simulink model "TP_CFO_Based_PP_pwm_mode"  (R2023b)
settings: Solver=ode4  StartTime=0.0  StopTime=inf  FixedStep=1/500  RelTol=1e-3  EnableMultiTasking=on
values from neighbouring files (symbols this model uses):
  home = [0.45;0;0.49]    [Params.m]
  K1 = [wc1^2,  2*xi1*wc1 - a1_1]    [Params.m]
  K2 = [wc2^2,  2*xi2*wc2 - a1_2]    [Params.m]
  K3 = [wc3^2,  2*xi3*wc3 - a1_3]    [Params.m]
  K4 = [wc4^2,  2*xi4*wc4 - a1_4]    [Params.m]
  pick = [0.66;0;0.3]    [Params.m]
  Place = [-0.425;0.5;0.35]    [Params.m]
undefined symbols (not defined in the file or in its folder): HIL
libraries: quarc_library x6
settings Model: ExtModeTrigDuration=10000  Creator=fvranes  LastModifiedBy=robot
settings SolverCC: AlgebraicLoopSolver=TrustRegion  PositivePriorityOrder=on
settings DataIOCC: ReturnWorkspaceOutputs=off
settings DebuggingCC: UnderspecifiedInitializationDetection=Classic  MergeDetectMultiDrivingBlocksExec=none  UnconnectedInputMsg=warning  UnconnectedOutputMsg=warning  UnconnectedLineMsg=warning
settings ModelReferenceCC: EnableRefExpFcnMdlSchedulingChecks=on  PropagateSignalLabelsOutOfModel=off
settings SFSimCC: CustomCodeUndefinedFunction=UseInterfaceOnly
settings RTWCC: Description=QUARC Win64 Target Using Toolchain  SystemTargetFile=quarc_win64.tlc  Toolchain=QUARC win64 | nmake (64-bit Windows)  BuildConfiguration=Faster Runs
settings STFCustomTargetCC: ConcurrentExecutionCompliant=on  GRTInterface=on  UseToolchainInfoCompliant=on  SystemTargetFile=quarc_win64.tlc
settings GRTTargetCC: ParMdlRefBuildCompliant=off  CompOptLevelCompliant=off  CombineOutputUpdateFcns=off  MatFileLogging=off  CPPClassGenCompliant=off  GRTInterface=on  ExtMode=on  ExtModeMexFile=quarc_comm

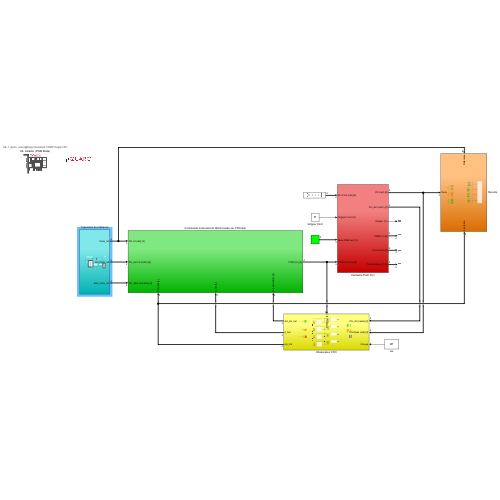
[thumbnail: Simulink's stored preview of the top-level diagram]
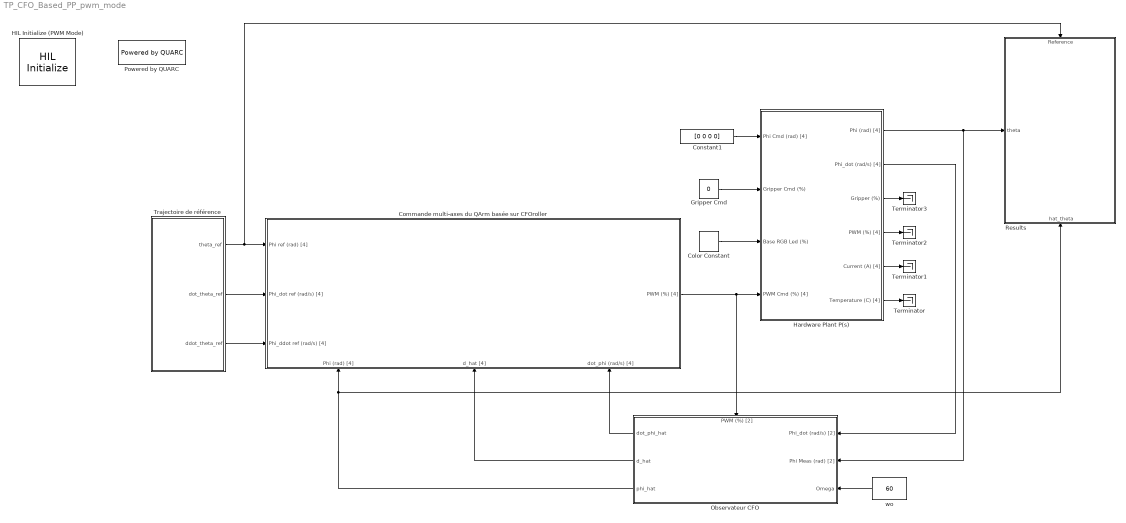
== system TP_CFO_Based_PP_pwm_mode ==
  Color Constant : quarc_library/Sources/Signals/Color Constant  color=[0 1 0]
      settings: SourceProductName=QUARC Targets
  Commande multi-axes du QArm basée sur CFOroller : Subsystem
      settings: PortSchema="{\"entries\":[{\"content\":{\"sides\":[{\"content\":{\"connectorIds\":[\"In1\",\"In2\",\"In3\"]},\"type\":\"ConnectorPlacement.EquallySpacedRectSide\",\"uuid\":\"25f6ea6f-3d46-46f3-9fc0-0185d57d9b43\"},{\"content\":{\"connectorIds\":[\"Out1\"],\"side\":\"RIGHT\"},\"type\":\"ConnectorPlacement.EquallySpacedRectSide\",\"uuid\":\"b6cf073e-ca4c-464e-b4e1-9442ca1008e1\"},{\"content\":{\"side\":\"TOP\"},\"type\":\"ConnectorPlacement.EquallySpacedRectSide\",\"uuid\":\"ffe5b829-7032-4458-83f6-b2e187a076e4\"},{\"content\":{\"connectorIds\":[\"In4\",\"In5\",\"In6\"],\"side\":\"BOTTOM\"},\"type\":\"ConnectorPlacement.EquallySpacedRectSide\",\"uuid\":\"4b5216bb-7b32-4753-9657-18d8be37116d\"}]},\"type\":\"ConnectorPlacement.EquallySpacedConnector\",\"uuid\":\"b7eb2212-47e7-4fcd-9e73-fc098706b9d4\"}],\"packageUris\":[\"http://schema.mathworks.com/mf0/Connector/R2020b\"],\"version\":\"1.0\"}"
  Constant1 : Constant  Value=[0 0 0 0]
  Gripper Cmd : Constant  Value=0
  HIL Initialize (PWM Mode) : quarc_library/Data Acquisition/Generic/Configuration/HIL Initialize  object_name=HIL-1  board_type=qarm_usb  board_number=0@tcpip://localhost:18900?nagle='off'  board_options=j0_mode=1;j1_mode=1;j2_mode=1;j3_mode=1;gripper_mode=0;  exclusive=off  active=on  hardware_clocks=[0]  clock_modes=[]  initial_clock_frequencies=[]  set_clock_params_at_start=off  set_clock_params_at_switch_in=off  set_clock_frequencies_at_start=off  set_clock_frequencies_at_switch_in=off  analog_input_channels=[5:9]  analog_input_configurations=[]  analog_input_maximums=[]  analog_input_minimums=[]  set_analog_input_params_at_start=off  set_analog_input_params_at_switch_in=off  analog_output_channels=[]  analog_output_maximums=inf  analog_output_minimums=-inf  initial_analog_outputs=[0]  final_analog_outputs=[0]  watchdog_analog_outputs=[]  set_analog_output_params_at_start=off  set_analog_output_params_at_switch_in=off  set_analog_outputs_at_start=off  set_analog_outputs_at_switch_in=off  set_analog_outputs_at_terminate=off  set_analog_outputs_at_switch_out=off  set_analog_outputs_on_watchdog=off  digital_input_channels=[]  digital_output_channels=[]  digital_output_configuration=[]  initial_digital_outputs=[0]  final_digital_outputs=[0]  watchdog_digital_outputs=[0]  set_digital_output_params_at_start=off  set_digital_output_params_at_switch_in=off  set_digital_outputs_at_start=off  set_digital_outputs_at_switch_in=off  set_digital_outputs_at_terminate=off  set_digital_outputs_at_switch_out=off  set_digital_outputs_on_watchdog=off  encoder_channels=[]  quadrature=[]  encoder_filter_frequency=[]  initial_encoder_counts=[]  set_encoder_params_at_start=off  set_encoder_params_at_switch_in=off  set_encoder_counts_at_start=off  set_encoder_counts_at_switch_in=off  pwm_channels=[]  pwm_modes=[]  pwm_frequency=[]  pwm_configuration=[]  pwm_alignment=[]  pwm_polarity=[]  pwm_leading_deadband=[]  pwm_trailing_deadband=[]  initial_pwm_outputs=[]  final_pwm_outputs=[]  watchdog_pwm_outputs=[]  set_pwm_params_at_start=off  set_pwm_params_at_switch_in=off  set_pwm_outputs_at_start=off  set_pwm_outputs_at_switch_in=off  set_pwm_outputs_at_terminate=off  set_pwm_outputs_at_switch_out=off  set_pwm_outputs_on_watchdog=off  other_output_channels=[1000:1004 11000:11003 11005:11007]  initial_other_outputs=[zeros(1,9), ones(1,3)]  final_other_outputs=[zeros(1,9), ones(1,3)]  watchdog_other_outputs=zeros(1,12)  set_other_outputs_at_start=off  set_other_outputs_at_switch_in=off  set_other_outputs_at_terminate=on  set_other_outputs_at_switch_out=off  set_other_outputs_on_watchdog=off
  Hardware Plant P(s) : Subsystem
  Observateur CFO : Subsystem
      settings: PortSchema="{\"entries\":[{\"content\":{\"sides\":[{\"content\":{\"connectorIds\":[\"Out1\",\"Out2\",\"Out3\"]},\"type\":\"ConnectorPlacement.EquallySpacedRectSide\",\"uuid\":\"b1ac645d-9d1e-4f6e-bc61-28976872a690\"},{\"content\":{\"connectorIds\":[\"In2\",\"In3\",\"In4\"],\"side\":\"RIGHT\"},\"type\":\"ConnectorPlacement.EquallySpacedRectSide\",\"uuid\":\"7e59dcac-6a8e-4444-81db-3f14db76565a\"},{\"content\":{\"connectorIds\":[\"In1\"],\"side\":\"TOP\"},\"type\":\"ConnectorPlacement.EquallySpacedRectSide\",\"uuid\":\"ce092a22-ec44-4e1c-8718-a0a100faa11b\"}]},\"type\":\"ConnectorPlacement.EquallySpacedConnector\",\"uuid\":\"dc8234ad-9229-4c64-a6ff-80b8db3f41cc\"}],\"packageUris\":[\"http://schema.mathworks.com/mf0/Connector/R2020b\"],\"version\":\"1.0\"}"
  Powered by QUARC : quarc_library/Logos/Powered by QUARC
  Results : Subsystem
      settings: PortSchema="{\"entries\":[{\"content\":{\"sides\":[{\"content\":{\"connectorIds\":[\"In1\"]},\"type\":\"ConnectorPlacement.EquallySpacedRectSide\",\"uuid\":\"fa6fdd80-9ba7-487b-8585-3ea4afe8c15a\"},{\"content\":{\"side\":\"RIGHT\"},\"type\":\"ConnectorPlacement.EquallySpacedRectSide\",\"uuid\":\"3312bcac-8289-413d-bf87-6a8d7db3217e\"},{\"content\":{\"connectorIds\":[\"In2\"],\"side\":\"TOP\"},\"type\":\"ConnectorPlacement.EquallySpacedRectSide\",\"uuid\":\"0731ee27-fa4b-422b-b333-a0e403238348\"},{\"content\":{\"connectorIds\":[\"In3\"],\"side\":\"BOTTOM\"},\"type\":\"ConnectorPlacement.EquallySpacedRectSide\",\"uuid\":\"d410c791-6845-40d9-b869-911e609371ee\"}]},\"type\":\"ConnectorPlacement.EquallySpacedConnector\",\"uuid\":\"747f7da3-1a68-4a17-a06e-f94e78aaaccb\"}],\"packageUris\":[\"http://schema.mathworks.com/mf0/Connector/R2020b\"],\"version\":\"1.0\"}"
  Terminator{,1..3} (4 alike) : Terminator
  Trajectoire de référence : Subsystem
  wo : Constant  Value=60
  wires:
  Color Constant/1 -> Hardware Plant P(s)/3(Base RGB Led (%))
  Hardware Plant P(s)/1(Phi (rad) [4]) -> Observateur CFO/3(Phi Meas (rad) [2]), Results/1(theta)
  Commande multi-axes du QArm basée sur CFOroller/1(PWM (%) [4]) -> Observateur CFO/1(PWM (%) [2]), Hardware Plant P(s)/4(PWM Cmd (%) [4])
  Constant1/1 -> Hardware Plant P(s)/1(Phi Cmd (rad) [4])
  wo/1 -> Observateur CFO/4(Omega)
  Trajectoire de référence/1(theta_ref) -> Commande multi-axes du QArm basée sur CFOroller/1(Phi ref (rad) [4]), Results/2(Reference)
  Trajectoire de référence/3(ddot_theta_ref) -> Commande multi-axes du QArm basée sur CFOroller/3(Phi_ddot ref (rad/s) [4])
  Trajectoire de référence/2(dot_theta_ref) -> Commande multi-axes du QArm basée sur CFOroller/2(Phi_dot ref (rad/s) [4])
  Hardware Plant P(s)/6(Temperature (C) [4]) -> Terminator/1
  Hardware Plant P(s)/5(Current (A) [4]) -> Terminator1/1
  Hardware Plant P(s)/4(PWM (%) [4]) -> Terminator2/1
  Hardware Plant P(s)/3(Gripper (%)) -> Terminator3/1
  Hardware Plant P(s)/2(Phi_dot (rad/s) [4]) -> Observateur CFO/2(Phi_dot (rad/s) [2])
  Gripper Cmd/1 -> Hardware Plant P(s)/2(Gripper Cmd (%))
  Observateur CFO/1(dot_phi_hat) -> Commande multi-axes du QArm basée sur CFOroller/6(dot_phi (rad/s) [4])
  Observateur CFO/2("d_hat ") -> Commande multi-axes du QArm basée sur CFOroller/5(d_hat [4])
  Observateur CFO/3(phi_hat) -> Commande multi-axes du QArm basée sur CFOroller/4(Phi (rad) [4]), Results/3(hat_theta)

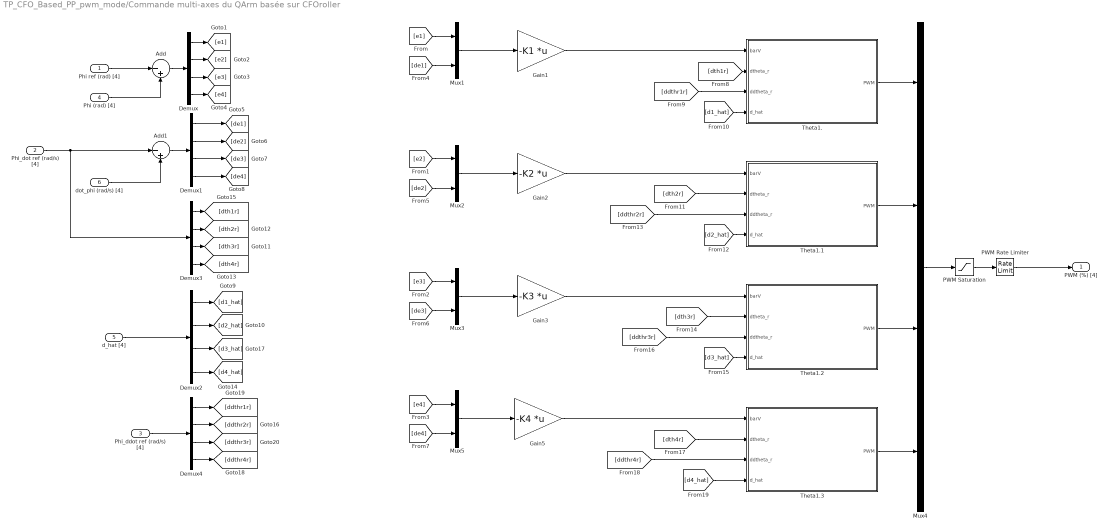
== system TP_CFO_Based_PP_pwm_mode/Commande multi-axes du QArm basée sur CFOroller ==
  Phi ref (rad) [4] : Inport
  Phi_dot ref (rad/s) [4] : Inport  Port=2
  Phi_ddot ref (rad/s) [4] : Inport  Port=3
  Phi (rad) [4] : Inport  Port=4
  d_hat [4] : Inport  Port=5
  dot_phi (rad/s) [4] : Inport  Port=6
  Add : Sum  Inputs=|-+
  Add1 : Sum  Inputs=|-+
  Demux{,1..4} (5 alike) : Demux
  Gain1 : Gain  Gain=-K1  Multiplication=Matrix(K*u)
  Gain2 : Gain  Gain=-K2  Multiplication=Matrix(K*u)
  Gain3 : Gain  Gain=-K3  Multiplication=Matrix(K*u)
  Gain5 : Gain  Gain=-K4  Multiplication=Matrix(K*u)
  Mux{1..3,5} (4 alike) : Mux  Inputs=2
  Mux4 : Mux
  PWM Rate Limiter : RateLimiter  RisingSlewLimit=0.5*[2 2 2 2]  FallingSlewLimit=0.5*[-2 -2 -2 -2]  SampleTimeMode=inherited
  PWM Saturation : Saturate  UpperLimit=[1 1 1 1]  LowerLimit=[-1 -1 -1 -1]
  Theta1. : MATLAB Function  TreatAsAtomicUnit=on
  Theta1.1 : MATLAB Function  TreatAsAtomicUnit=on
  Theta1.2 : MATLAB Function  TreatAsAtomicUnit=on
  Theta1.3 : MATLAB Function  TreatAsAtomicUnit=on
  PWM (%) [4] : Outport  VectorParamsAs1DForOutWhenUnconnected=off
  wires:
  PWM Saturation/1 -> PWM Rate Limiter/1
  PWM Rate Limiter/1 -> PWM (%) [4]/1
  [e1] -> Mux1/1
  Add1/1 -> Demux1/1
  Phi (rad) [4]/1 -> Add/2
  Phi_ddot ref (rad/s) [4]/1 -> Demux4/1
  [e2] -> Mux2/1
  [de2] -> Mux2/2
  Phi_dot ref (rad/s) [4]/1 -> Demux3/1, Add1/1
  [d2_hat] -> Theta1.1/4(d_hat)
  dot_phi (rad/s) [4]/1 -> Add1/2
  [de1] -> Mux1/2
  Add/1 -> Demux/1
  Phi ref (rad) [4]/1 -> Add/1
  Mux4/1 -> PWM Saturation/1
  d_hat [4]/1 -> Demux2/1
  [d1_hat] -> Theta1./4(d_hat)
  Theta1./1(PWM) -> Mux4/1
  Theta1.1/1(PWM) -> Mux4/2
  Demux/1 -> [e1]
  Demux/2 -> [e2]
  Demux3/1 -> [dth1r]
  Demux3/2 -> [dth2r]
  Demux2/1 -> [d1_hat]
  Demux2/2 -> [d2_hat]
  Demux4/1 -> [ddthr1r]
  Demux4/2 -> [ddthr2r]
  Demux/3 -> [e3]
  Demux/4 -> [e4]
  Demux1/1 -> [de1]
  Demux1/2 -> [de2]
  Demux1/3 -> [de3]
  Demux1/4 -> [de4]
  Demux3/3 -> [dth3r]
  Demux3/4 -> [dth4r]
  Demux2/3 -> [d3_hat]
  Demux2/4 -> [d4_hat]
  Demux4/3 -> [ddthr3r]
  Demux4/4 -> [ddthr4r]
  Theta1.3/1(PWM) -> Mux4/4
  Theta1.2/1(PWM) -> Mux4/3
  [d3_hat] -> Theta1.2/4(d_hat)
  [de3] -> Mux3/2
  [de4] -> Mux5/2
  [e4] -> Mux5/1
  [e3] -> Mux3/1
  [dth1r] -> Theta1./2(dtheta_r)
  [ddthr1r] -> Theta1./3(ddtheta_r)
  [dth2r] -> Theta1.1/2(dtheta_r)
  [ddthr2r] -> Theta1.1/3(ddtheta_r)
  [dth3r] -> Theta1.2/2(dtheta_r)
  [ddthr3r] -> Theta1.2/3(ddtheta_r)
  [dth4r] -> Theta1.3/2(dtheta_r)
  [ddthr4r] -> Theta1.3/3(ddtheta_r)
  [d4_hat] -> Theta1.3/4(d_hat)
  Gain1/1 -> Theta1./1(barV)
  Gain2/1 -> Theta1.1/1(barV)
  Gain3/1 -> Theta1.2/1(barV)
  Gain5/1 -> Theta1.3/1(barV)
  Mux5/1 -> Gain5/1
  Mux3/1 -> Gain3/1
  Mux2/1 -> Gain2/1
  Mux1/1 -> Gain1/1

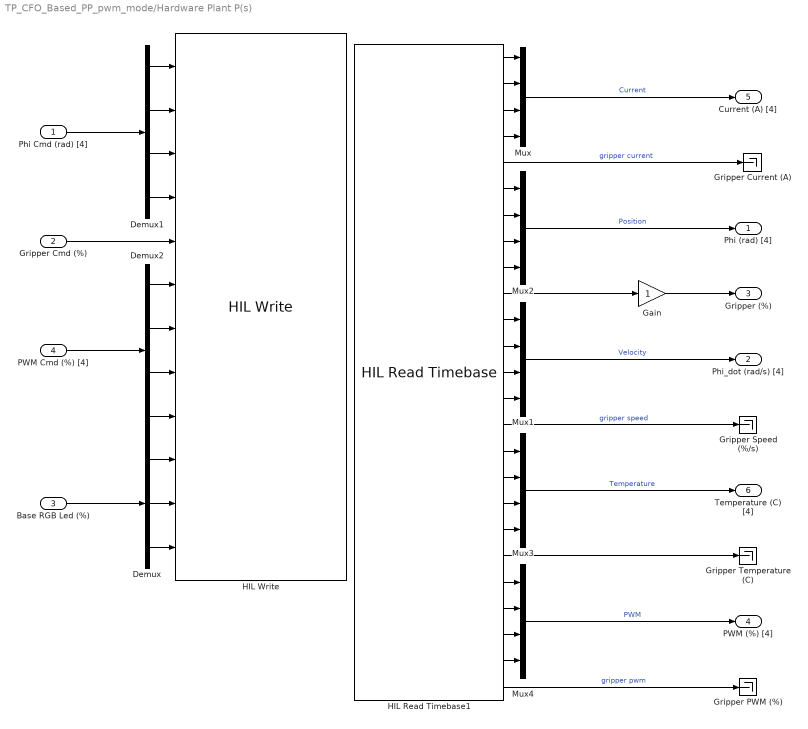
== system TP_CFO_Based_PP_pwm_mode/Hardware Plant P(s) ==
  Phi Cmd (rad) [4] : Inport
  Gripper Cmd (%) : Inport  Port=2
  Base RGB Led (%) : Inport  Port=3
  PWM Cmd (%) [4] : Inport  Port=4
  Demux : Demux  Outputs=3
  Demux1 : Demux
  Demux2 : Demux
  Gain : Gain
  Gripper Current (A) : Terminator
  Gripper PWM (%) : Terminator
  Gripper Speed (%/s) : Terminator
  Gripper Temperature (C) : Terminator
  HIL Read Timebase1 : quarc_library/Data Acquisition/Generic/Timebases/HIL Read Timebase  object_name=HIL-1  clock=0  analog_channels=[5:9]  encoder_channels=[]  digital_channels=[]  other_channels=[1000:1004 3000:3004 10000:10004 11000:11004]  active=on  vector_output=off  data_type_mode=Inherit via back propagation  encoder_data_type=double  digital_data_type=boolean  overflow_mode=Synchronize (for simulated cards only)  samples_in_buffer=1
  HIL Write : quarc_library/Data Acquisition/Generic/Immediate I//O/HIL Write  object_name=HIL-1  analog_channels=[]  pwm_channels=[]  digital_channels=[]  other_channels=[1000:1004 11000:11003 11005:11007]  sample_time=-1  active=on  vector_input=off
  Mux{,1..4} (5 alike) : Mux
  Phi (rad) [4] : Outport  VectorParamsAs1DForOutWhenUnconnected=off
  Phi_dot (rad/s) [4] : Outport  Port=2  VectorParamsAs1DForOutWhenUnconnected=off
  Gripper (%) : Outport  Port=3  VectorParamsAs1DForOutWhenUnconnected=off
  PWM (%) [4] : Outport  Port=4  VectorParamsAs1DForOutWhenUnconnected=off
  Current (A) [4] : Outport  Port=5  VectorParamsAs1DForOutWhenUnconnected=off
  Temperature (C) [4] : Outport  Port=6  VectorParamsAs1DForOutWhenUnconnected=off
  wires:
  HIL Read Timebase1/14 -> Mux1/4
  HIL Read Timebase1/9 -> Mux2/4
  HIL Read Timebase1/6 -> Mux2/1
  HIL Read Timebase1/18 -> Mux3/3
  HIL Read Timebase1/8 -> Mux2/3
  HIL Read Timebase1/12 -> Mux1/2
  HIL Read Timebase1/4 -> Mux/4
  HIL Read Timebase1/7 -> Mux2/2
  HIL Read Timebase1/5 -> Gripper Current (A)/1  "gripper current"
  HIL Read Timebase1/15 -> Gripper Speed (%/s)/1  "gripper speed"
  Demux/3 -> HIL Write/12
  HIL Read Timebase1/3 -> Mux/3
  HIL Read Timebase1/17 -> Mux3/2
  HIL Read Timebase1/16 -> Mux3/1
  HIL Read Timebase1/11 -> Mux1/1
  Demux/1 -> HIL Write/10
  HIL Read Timebase1/19 -> Mux3/4
  Demux/2 -> HIL Write/11
  HIL Read Timebase1/13 -> Mux1/3
  HIL Read Timebase1/2 -> Mux/2
  HIL Read Timebase1/1 -> Mux/1
  HIL Read Timebase1/20 -> Gripper Temperature (C)/1
  Mux/1 -> Current (A) [4]/1  "Current"
  Mux1/1 -> Phi_dot (rad/s) [4]/1  "Velocity"
  Mux3/1 -> Temperature (C) [4]/1  "Temperature"
  Base RGB Led (%)/1 -> Demux/1
  Demux1/1 -> HIL Write/1
  Demux1/2 -> HIL Write/2
  Demux1/3 -> HIL Write/3
  Demux1/4 -> HIL Write/4
  Phi Cmd (rad) [4]/1 -> Demux1/1
  PWM Cmd (%) [4]/1 -> Demux2/1
  Demux2/1 -> HIL Write/6
  Demux2/2 -> HIL Write/7
  Demux2/3 -> HIL Write/8
  Demux2/4 -> HIL Write/9
  Mux2/1 -> Phi (rad) [4]/1  "Position"
  HIL Read Timebase1/21 -> Mux4/1
  HIL Read Timebase1/22 -> Mux4/2
  HIL Read Timebase1/23 -> Mux4/3
  HIL Read Timebase1/24 -> Mux4/4
  HIL Read Timebase1/25 -> Gripper PWM (%)/1  "gripper pwm"
  Mux4/1 -> PWM (%) [4]/1  "PWM"
  HIL Read Timebase1/10 -> Gain/1
  Gain/1 -> Gripper (%)/1
  Gripper Cmd (%)/1 -> HIL Write/5

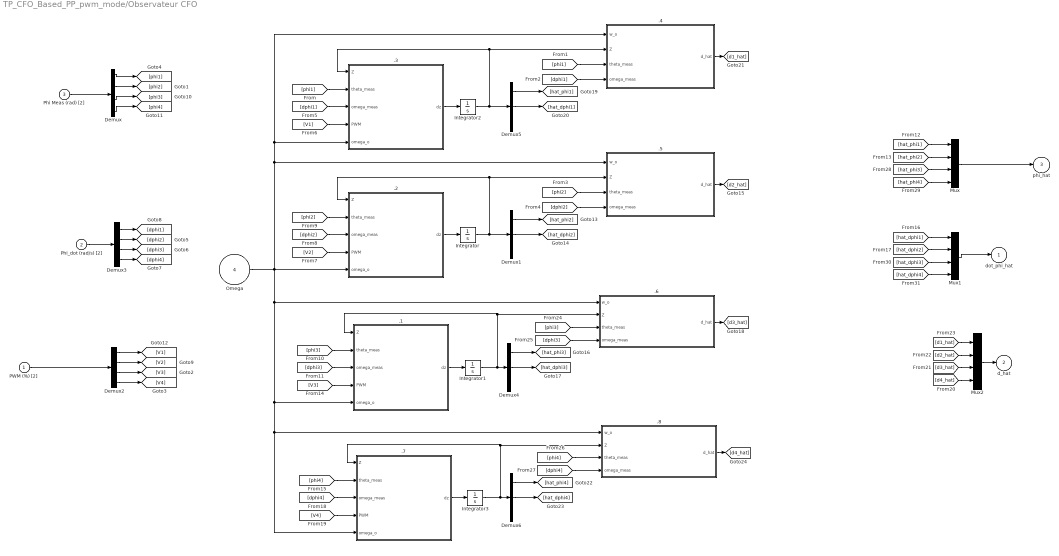
== system TP_CFO_Based_PP_pwm_mode/Observateur CFO ==
  PWM (%) [2] : Inport
  Phi_dot (rad/s) [2] : Inport  Port=2
  Phi Meas (rad) [2] : Inport  Port=3
  Omega : Inport  Port=4
  .1 : MATLAB Function  TreatAsAtomicUnit=on
  .2 : MATLAB Function  TreatAsAtomicUnit=on
  .3 : MATLAB Function  TreatAsAtomicUnit=on
  .4 : MATLAB Function  TreatAsAtomicUnit=on
  .5 : MATLAB Function  TreatAsAtomicUnit=on
  .6 : MATLAB Function  TreatAsAtomicUnit=on
  .7 : MATLAB Function  TreatAsAtomicUnit=on
  .8 : MATLAB Function  TreatAsAtomicUnit=on
  Demux : Demux
  Demux{1,4..6} (4 alike) : Demux  Outputs=3
  Demux2 : Demux
  Demux3 : Demux
  Integrator : Integrator  InitialCondition=[3.5*10^-3 0 0]
  Integrator1 : Integrator  InitialCondition=[5*10^-3 0 0]
  Integrator2 : Integrator  InitialCondition=[0 0 0]
  Integrator3 : Integrator  InitialCondition=[0 0 0]
  Mux : Mux
  Mux1 : Mux
  Mux2 : Mux
  dot_phi_hat : Outport
  "d_hat " : Outport  Port=2
  phi_hat : Outport  Port=3
  wires:
  .2/1(dz) -> Integrator/1
  Integrator/1 -> .5/2(Z), .2/1(Z), Demux1/1
  [V2] -> .2/4(PWM)
  Phi Meas (rad) [2]/1 -> Demux/1
  Phi_dot (rad/s) [2]/1 -> Demux3/1
  Demux/1 -> [phi1]
  Demux/2 -> [phi2]
  Demux3/1 -> [dphi1]
  Demux3/2 -> [dphi2]
  Demux2/1 -> [V1]
  Demux2/2 -> [V2]
  [phi2] -> .2/2(theta_meas)
  [dphi2] -> .2/3(omega_meas)
  Demux1/1 -> [hat_phi2]
  Demux1/2 -> [hat_dphi2]
  [dphi3] -> .1/3(omega_meas)
  [phi3] -> .1/2(theta_meas)
  [V3] -> .1/4(PWM)
  Integrator1/1 -> .1/1(Z), .6/2(Z), Demux4/1
  .1/1(dz) -> Integrator1/1
  Mux/1 -> phi_hat/1
  Mux1/1 -> dot_phi_hat/1
  Mux2/1 -> "d_hat "/1
  [hat_phi1] -> Mux/1
  [hat_phi2] -> Mux/2
  [hat_dphi1] -> Mux1/1
  [hat_dphi2] -> Mux1/2
  [d1_hat] -> Mux2/1
  [d2_hat] -> Mux2/2
  Demux4/1 -> [hat_phi3]
  Demux4/2 -> [hat_dphi3]
  [phi2] -> .5/3(theta_meas)
  [dphi2] -> .5/4(omega_meas)
  .5/1(d_hat) -> [d2_hat]
  [phi3] -> .6/3(theta_meas)
  [dphi3] -> .6/4(omega_meas)
  .6/1(d_hat) -> [d3_hat]
  Demux2/4 -> [V4]
  Demux2/3 -> [V3]
  Demux3/3 -> [dphi3]
  Demux3/4 -> [dphi4]
  Demux/3 -> [phi3]
  Demux/4 -> [phi4]
  .4/1(d_hat) -> [d1_hat]
  Omega/1 -> .4/1(w_o), .3/5(omega_o), .5/1(w_o), .2/5(omega_o), .6/1(w_o), .7/5(omega_o), .8/1(w_o), .1/5(omega_o)
  Demux5/2 -> [hat_dphi1]
  Demux5/1 -> [hat_phi1]
  [dphi1] -> .3/3(omega_meas)
  [phi1] -> .3/2(theta_meas)
  [V1] -> .3/4(PWM)
  Integrator2/1 -> Demux5/1, .3/1(Z), .4/2(Z)
  .3/1(dz) -> Integrator2/1
  .8/1(d_hat) -> [d4_hat]
  [dphi4] -> .8/4(omega_meas)
  [phi4] -> .8/3(theta_meas)
  Demux6/2 -> [hat_dphi4]
  Demux6/1 -> [hat_phi4]
  .7/1(dz) -> Integrator3/1
  Integrator3/1 -> Demux6/1, .8/2(Z), .7/1(Z)
  [V4] -> .7/4(PWM)
  [phi4] -> .7/2(theta_meas)
  [dphi4] -> .7/3(omega_meas)
  [d3_hat] -> Mux2/3
  [d4_hat] -> Mux2/4
  [hat_phi3] -> Mux/3
  [hat_phi4] -> Mux/4
  [hat_dphi3] -> Mux1/3
  [hat_dphi4] -> Mux1/4
  PWM (%) [2]/1 -> Demux2/1
  [phi1] -> .4/3(theta_meas)
  [dphi1] -> .4/4(omega_meas)

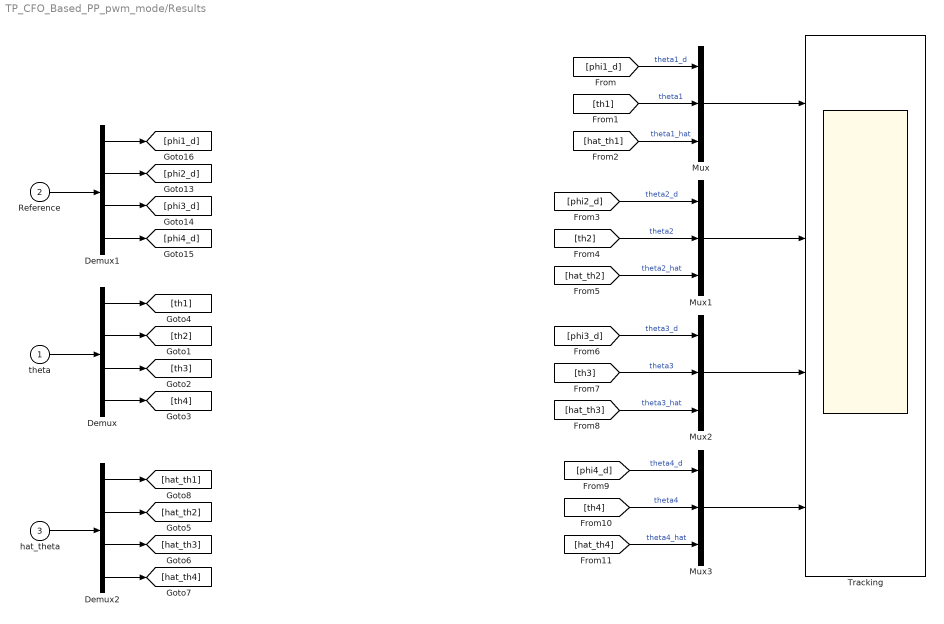
== system TP_CFO_Based_PP_pwm_mode/Results ==
  theta : Inport
  Reference : Inport  Port=2
  hat_theta : Inport  Port=3
  Demux : Demux
  Demux1 : Demux
  Demux2 : Demux
  Mux{,1..3} (4 alike) : Mux  Inputs=3
  Tracking : Scope  NumInputPorts=4
  wires:
  Mux/1 -> Tracking/1
  Demux/3 -> [th3]
  theta/1 -> Demux/1
  Demux/4 -> [th4]
  Demux/2 -> [th2]
  Demux/1 -> [th1]
  Demux1/1 -> [phi1_d]
  Demux1/2 -> [phi2_d]
  Demux1/4 -> [phi4_d]
  Reference/1 -> Demux1/1
  Demux1/3 -> [phi3_d]
  Demux2/1 -> [hat_th1]
  Demux2/2 -> [hat_th2]
  Demux2/4 -> [hat_th4]
  hat_theta/1 -> Demux2/1
  Demux2/3 -> [hat_th3]
  [phi1_d] -> Mux/1  "theta1_d"
  [th1] -> Mux/2  "theta1"
  [hat_th1] -> Mux/3  "theta1_hat"
  Mux1/1 -> Tracking/2
  Mux2/1 -> Tracking/3
  Mux3/1 -> Tracking/4
  [phi2_d] -> Mux1/1  "theta2_d"
  [th2] -> Mux1/2  "theta2"
  [hat_th2] -> Mux1/3  "theta2_hat"
  [phi3_d] -> Mux2/1  "theta3_d"
  [th3] -> Mux2/2  "theta3"
  [hat_th3] -> Mux2/3  "theta3_hat"
  [phi4_d] -> Mux3/1  "theta4_d"
  [th4] -> Mux3/2  "theta4"
  [hat_th4] -> Mux3/3  "theta4_hat"

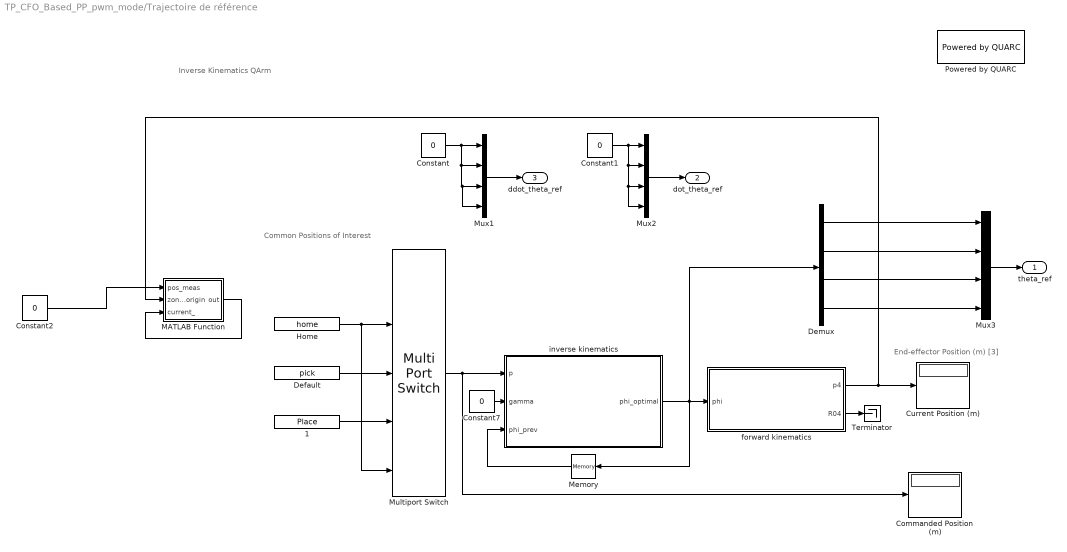
== system TP_CFO_Based_PP_pwm_mode/Trajectoire de référence ==
  note: Inverse Kinematics
      | QArm
  note: End-effector
      | Position (m) [3]
  note: Common Positions of Interest
  1 : Constant  Value=Place
  Commanded Position (m) : Display
  Constant{,1..2,7} (4 alike) : Constant  Value=0
  Current Position (m) : Display
  Default : Constant  Value=pick
  Demux : Demux
  Home : Constant  Value=home
  MATLAB Function : MATLAB Function  TreatAsAtomicUnit=on
  Memory : Memory  InitialCondition=[0 0 0 0]
  Multiport Switch : MultiPortSwitch  DataPortForDefault=Additional data port  SaturateOnIntegerOverflow=off  InputSameDT=off
  Mux1 : Mux
  Mux2 : Mux
  Mux3 : Mux
  Powered by QUARC : quarc_library/Logos/Powered by QUARC
  Terminator : Terminator
  forward kinematics : MATLAB Function  TreatAsAtomicUnit=on
  inverse kinematics : MATLAB Function  TreatAsAtomicUnit=on
  theta_ref : Outport
  dot_theta_ref : Outport  Port=2
  ddot_theta_ref : Outport  Port=3
  wires:
  Constant/1 -> Mux1/4, Mux1/3, Mux1/2, Mux1/1
  Constant1/1 -> Mux2/4, Mux2/3, Mux2/2, Mux2/1
  Mux2/1 -> dot_theta_ref/1
  Mux1/1 -> ddot_theta_ref/1
  Constant7/1 -> inverse kinematics/2(gamma)
  inverse kinematics/1(phi_optimal) -> Demux/1, Memory/1, forward kinematics/1(phi)
  1/1 -> Multiport Switch/4
  Multiport Switch/1 -> Commanded Position (m)/1, inverse kinematics/1(p)
  forward kinematics/1(p4) -> MATLAB Function/2(zone_origin), Current Position (m)/1
  Home/1 -> Multiport Switch/5, Multiport Switch/2
  Default/1 -> Multiport Switch/3
  forward kinematics/2(R04) -> Terminator/1
  Memory/1 -> inverse kinematics/3(phi_prev)
  Demux/1 -> Mux3/1
  Demux/4 -> Mux3/4
  Demux/3 -> Mux3/3
  Demux/2 -> Mux3/2
  Mux3/1 -> theta_ref/1
  Constant2/1 -> MATLAB Function/1(pos_meas)
  MATLAB Function/1(out) -> MATLAB Function/3(current_)

== matlab function TP_CFO_Based_PP_pwm_mode/Observateur CFO/.5 ==
  data: w_o input; Z input; theta_meas input; omega_meas input; d_hat output
function d_hat  = tau_tot_hat_joint1(w_o,Z, theta_meas, omega_meas)


z1 = Z(1); z2 = Z(2); z3 = Z(3);


%% Erreurs d'observation
e_theta = theta_meas - z1;
e_omega = omega_meas - z2;

%% Gains CFO
l1 = 9*w_o;
l2 = 12*w_o*w_o;

%% Terme de correction
Le = l2*e_theta + l1*e_omega;

d_hat = Le + z3;
end

== matlab function TP_CFO_Based_PP_pwm_mode/Observateur CFO/.6 ==
  data: w_o input; Z input; theta_meas input; omega_meas input; d_hat output
function d_hat = d_hat_joint3(w_o, Z, theta_meas, omega_meas)

z1 = Z(1);
z2 = Z(2);
z3 = Z(3);



%% Erreurs d'observation
e_theta = theta_meas - z1;
e_omega = omega_meas - z2;

%% Gains CFO
l1 = 9*w_o;
l2 = 12*w_o*w_o;

%% Terme de correction
Le = l2*e_theta + l1*e_omega;

d_hat = Le + z3;
end

== matlab function TP_CFO_Based_PP_pwm_mode/Observateur CFO/.3 ==
  data: Z input; theta_meas input; omega_meas input; PWM input; dz output; omega_o input
function dz = cfo_obs_joint1(Z, theta_meas, omega_meas, PWM, omega_o)

% CFO - Joint 1
V = 12*PWM;
%% Etats observateur
z1 = Z(1);      % theta_hat
z2 = Z(2);      % omega_hat
z3 = Z(3);      % etat interne CFO

%% Parametres Joint 1
a0 = 23.4652;
a1 = 91.4161;

%% Erreurs d'observation
e_theta = theta_meas - z1;
e_omega = omega_meas - z2;

%% Gains CFO
l1 = 9*omega_o;
l2 = 12*omega_o*omega_o;
lambda = (4/3)*omega_o;

%% Terme de correction
Le = l2*e_theta + l1*e_omega;

%% Dynamique CFO
theta_point_hat = z2;
omega_point_hat = -a1*z2+a0*V+Le+z3;
z3_point = lambda * Le;

%% Sortie
dz = [theta_point_hat omega_point_hat z3_point];


end

== matlab function TP_CFO_Based_PP_pwm_mode/Observateur CFO/.4 ==
  data: w_o input; Z input; theta_meas input; omega_meas input; d_hat output
function d_hat = d_hat_joint2(w_o, Z, theta_meas, omega_meas)

z1 = Z(1);
z2 = Z(2);
z3 = Z(3);

%% Erreurs d'observation
e_theta = theta_meas - z1;
e_omega = omega_meas - z2;

%% Gains CFO
l1 = 9*w_o;
l2 = 12*w_o*w_o;

%% Terme de correction
Le = l2*e_theta + l1*e_omega;

d_hat = Le + z3;
end

== matlab function TP_CFO_Based_PP_pwm_mode/Observateur CFO/.7 ==
  data: Z input; theta_meas input; omega_meas input; PWM input; dz output; omega_o input
function dz = cfo_obs_joint4(Z, theta_meas, omega_meas, PWM, omega_o)

z1 = Z(1);
z2 = Z(2);
z3 = Z(3);

% Parametres locaux Joint 4
a0 = 271.48313954;
a1 = 671.78502879;

% PWM -> tension
V = 12*PWM;

%% Erreurs d'observation
e_theta = theta_meas - z1;
e_omega = omega_meas - z2;

%% Gains CFO
l1 = 9*omega_o;
l2 = 12*omega_o*omega_o;
lambda = (4/3)*omega_o;

%% Terme de correction
Le = l2*e_theta + l1*e_omega;

%% Dynamique CFO
theta_point_hat = z2;
omega_point_hat = -a1*z2+a0*V+Le+z3;
z3_point = lambda * Le;

%% Sortie
dz = [theta_point_hat omega_point_hat z3_point];


end

== matlab function TP_CFO_Based_PP_pwm_mode/Observateur CFO/.2 ==
  data: Z input; theta_meas input; omega_meas input; PWM input; dz output; omega_o input
function dz = cfo_obs_joint2(Z, theta_meas, omega_meas, PWM, omega_o)

z1 = Z(1);
z2 = Z(2);
z3 = Z(3);

% Parametres locaux Joint 2
a0 = 17.59887839;
a1 = 68.11562089;

% PWM -> tension
V = 12*PWM;

%% Erreurs d'observation
e_theta = theta_meas - z1;
e_omega = omega_meas - z2;

%% Gains CFO
l1 = 9*omega_o;
l2 = 12*omega_o*omega_o;
lambda = (4/3)*omega_o;

%% Terme de correction
Le = l2*e_theta + l1*e_omega;

%% Dynamique CFO
theta_point_hat = z2;
omega_point_hat = -a1*z2+a0*V+Le+z3;
z3_point = lambda * Le;

%% Sortie
dz = [theta_point_hat omega_point_hat z3_point];


end

== matlab function TP_CFO_Based_PP_pwm_mode/Observateur CFO/.8 ==
  data: w_o input; Z input; theta_meas input; omega_meas input; d_hat output
function d_hat = d_hat_joint4(w_o, Z, theta_meas, omega_meas)

z1 = Z(1);
z2 = Z(2);
z3 = Z(3);

%% Erreurs d'observation
e_theta = theta_meas - z1;
e_omega = omega_meas - z2;

%% Gains CFO
l1 = 9*w_o;
l2 = 12*w_o*w_o;

%% Terme de correction
Le = l2*e_theta + l1*e_omega;

d_hat = Le + z3;
end

== matlab function TP_CFO_Based_PP_pwm_mode/Commande multi-axes du QArm basée sur CFOroller/Theta1.1 ==
  data: barV input; dtheta_r input; ddtheta_r input; PWM output; d_hat input
function PWM = joint2_control(barV, dtheta_r, ddtheta_r, d_hat)

a0 = 17.59887839;
a1 = 68.11562089;

V = (barV-d_hat+a1*dtheta_r+ddtheta_r)/(a0);

% Saturation 
if V > 12
    V = 12;
elseif V < -12
    V = -12;
end

% Tension -> PWM
PWM = V/12;

end

== matlab function TP_CFO_Based_PP_pwm_mode/Commande multi-axes du QArm basée sur CFOroller/Theta1.2 ==
  data: barV input; dtheta_r input; ddtheta_r input; PWM output; d_hat input
function PWM = joint3_control(barV, dtheta_r, ddtheta_r, d_hat)

a0 = 23.46517119;
a1 = 93.20178023;

V = (barV-d_hat+a1*dtheta_r+ddtheta_r)/(a0);

if V > 12
    V = 12;
elseif V < -12
    V = -12;
end

PWM = V/12;

end

== matlab function TP_CFO_Based_PP_pwm_mode/Commande multi-axes du QArm basée sur CFOroller/Theta1. ==
  data: barV input; dtheta_r input; ddtheta_r input; PWM output; d_hat input
function PWM = joint1_control(barV, dtheta_r, ddtheta_r, d_hat)

%% Parametres Joint 1
a0 = 23.46517119;
a1 = 91.41606594;

%% Tension moteur
V = (barV-d_hat+a1*dtheta_r+ddtheta_r)/(a0);

%% Saturation 
if V > 12
    V = 12;
elseif V < -12
    V = -12;
end

%% Conversion tension -> PWM normalise
PWM = V/12;

end

== matlab function TP_CFO_Based_PP_pwm_mode/Commande multi-axes du QArm basée sur CFOroller/Theta1.3 ==
  data: barV input; dtheta_r input; ddtheta_r input; PWM output; d_hat input
function PWM = joint4_control(barV, dtheta_r, ddtheta_r, d_hat)

a0 = 271.48313954;
a1 = 671.78502879;

V = (barV-d_hat+a1*dtheta_r+ddtheta_r)/(a0);

if V > 12
    V = 12;
elseif V < -12
    V = -12;
end

PWM = V/12;

end

== matlab function TP_CFO_Based_PP_pwm_mode/Observateur CFO/.1 ==
  data: Z input; theta_meas input; omega_meas input; PWM input; dz output; omega_o input
function dz = cfo_obs_joint3(Z, theta_meas, omega_meas, PWM, omega_o)

z1 = Z(1);
z2 = Z(2);
z3 = Z(3);

% Parametres Joint 3
a0 = 23.46517119;
a1 = 93.20178023;

% PWM -> tension
V = 12*PWM;

%% Erreurs d'observation
e_theta = theta_meas - z1;
e_omega = omega_meas - z2;

%% Gains CFO
l1 = 9*omega_o;
l2 = 12*omega_o*omega_o;
lambda = (4/3)*omega_o;

%% Terme de correction
Le = l2*e_theta + l1*e_omega;

%% Dynamique CFO
theta_point_hat = z2;
omega_point_hat = -a1*z2+a0*V+Le+z3;
z3_point = lambda * Le;

%% Sortie
dz = [theta_point_hat omega_point_hat z3_point];
end

== matlab function TP_CFO_Based_PP_pwm_mode/Trajectoire de référence/forward kinematics ==
  data: phi input; p4 output; R04 output
function [p4, R04] = qarmForwardKinematics(phi)

%% QUANSER_ARM_FPK
% v 4.0 - 4th June 2020

% REFERENCE: 
% Chapter 3. Forward Kinematics
% Robot Dynamics and Control 
% Spong, Vidyasagar
% 1989

% INPUTS:
% phi     : Alternate joint angles vector 4 x 1

% OUTPUTS:
% p4      : End-effector frame {4} position vector expressed in base frame {0}
% R04     : rotation matrix from end-effector frame {4} to base frame {0}

%% Manipulator parameters:
L1 = 0.1400;
L2 = 0.3500;
L3 = 0.0500;
L4 = 0.2500;
L5 = 0.1500;

%% Alternate parameters
l1 = L1;
l2 = sqrt(L2^2 + L3^2);
l3 = L4 + L5;
beta = atan(L3/L2);

%% From phi space to theta space 
theta = phi;
theta(1) = phi(1);
theta(2) = phi(2) + beta - pi/2;
theta(3) = phi(3) - beta;
theta(4) = phi(4);

%% Transformation matrices for all frames:

% T{i-1}{i} = quanser_arm_DH(  a, alpha,  d,     theta );
        T01 = quanser_arm_DH(  0, -pi/2, l1,  theta(1) );
        T12 = quanser_arm_DH( l2,     0,  0,  theta(2) );
        T23 = quanser_arm_DH(  0, -pi/2,  0,  theta(3) );
        T34 = quanser_arm_DH(  0,     0, l3,  theta(4) );

        T02 = T01*T12;
        T03 = T02*T23;
        T04 = T03*T34;

%% Position of end-effector Transformation

% Extract the Position vector 
% p1   = T01(1:3,4);
% p2   = T02(1:3,4);
% p3   = T03(1:3,4);
p4   = T04(1:3,4);

% Extract the Rotation matrix
% R01 = T01(1:3,1:3);
% R02 = T02(1:3,1:3);
% R03 = T03(1:3,1:3);
R04 = T04(1:3,1:3);

end

function T = quanser_arm_DH(a,alpha,d,theta)

%% QUANSER_ARM_DH
% v 1.0 - 26th March 2019

% REFERENCE: 
% Chapter 3. Forward and Inverse Kinematics
% Robot Modeling and Control 
% Spong, Hutchinson, Vidyasagar
% 2006

% INPUTS:
% a       :   translation  : along : x_{i}   : from : z_{i-1} : to : z_{i}
% alpha   :      rotation  : about : x_{i}   : from : z_{i-1} : to : z_{i}
% d       :   translation  : along : z_{i-1} : from : x_{i-1} : to : x_{i}
% theta   :      rotation  : about : z_{i-1} : from : x_{i-1} : to : x_{i}
% NOTE: Standard DH Parameters

% OUTPUTS:
% T       : transformation                   : from :     {i} : to : {i-1}

%%
% Rotation Transformation about z axis by theta
T_R_z = [cos(theta) -sin(theta) 0 0;
         sin(theta)  cos(theta) 0 0;
                  0           0 1 0;
                  0           0 0 1];
     
% Translation Transformation along z axis by d
T_T_z = [1 0 0 0;
         0 1 0 0;
         0 0 1 d;
         0 0 0 1];

% Translation Transformation along x axis by a
T_T_x = [1 0 0 a;
         0 1 0 0;
         0 0 1 0;
         0 0 0 1];

% Rotation Transformation about x axis by alpha
T_R_x = [1          0           0 0;
         0 cos(alpha) -sin(alpha) 0;
         0 sin(alpha)  cos(alpha) 0;
         0          0           0 1];

% For a transformation FROM frame {i} TO frame {i-1}: A
T = T_R_z*T_T_z*T_T_x*T_R_x;

end

== matlab function TP_CFO_Based_PP_pwm_mode/Trajectoire de référence/inverse kinematics ==
  data: p input; gamma input; phi_optimal output; phi_prev input
function phi_optimal   = qarmInverseKinematics(p, gamma, phi_prev)

%% QUANSER_ARM_IPK
% v 4.0 - 4th June 2020

% REFERENCE: 
% Chapter 4. Inverse Kinematics
% Robot Dynamics and Control 
% Spong, Vidyasagar
% 1989

% INPUTS:
% p        : end-effector position vector expressed in base frame {0}
% gamma    : wrist rotation angle gamma

% OUTPUTS:
% phi_optimal : Best solution depending on phi_prev
% phi         : All four Inverse Kinematics solutions as a 4x4 matrix. 
%               Each col is a solution.

%% Manipulator parameters:
L1 = 0.1400;
L2 = 0.3500;
L3 = 0.0500;
L4 = 0.2500;
L5 = 0.1500;
beta = atan(L3/L2);

%% Alternate parameters
lambda1 = L1;
lambda2 = sqrt(L2^2 + L3^2);
lambda3 = L4 + L5;

%% Initialization
theta   = zeros(4, 4);
phi = zeros(4, 4);

%% Joint angle 2 and 3: 
% Equations:
    % lambda2 cos(theta2) + (-lambda3) sin(theta2 + theta3) = sqrt(x^2 + y^2)
    %   A     cos( 2    ) +     C      sin(   2   +    3  ) =    D
    
    % lambda2 sin(theta2) - (-lambda3) cos(theta2 + theta3) = lambda1 - z
    %   A     sin( 2    ) -     C      cos(   2   +    3  ) =    H

% Solution:
    A = lambda2;
    C = -lambda3;
    H =  lambda1 - p(3);
    D1 = -sqrt(p(1)^2 + p(2)^2);
    D2 = sqrt(p(1)^2 + p(2)^2);
    F = (D1^2 + H^2 - A^2 - C^2)/(2*A);

    theta(3,1) = 2*atan2( C + sqrt(C^2 - F^2) , F );
	theta(3,2) = 2*atan2( C - sqrt(C^2 - F^2) , F );
    theta(3,3) = 2*atan2( C + sqrt(C^2 - F^2) , F );
	theta(3,4) = 2*atan2( C - sqrt(C^2 - F^2) , F );

    M = A + C*sin(theta(3,1));
    N = -C*cos(theta(3,1));
    cos_term = (D1*M + H*N)/(M^2 + N^2);
    sin_term = (H - N*cos_term)/(M);
    theta(2,1) = atan2(sin_term, cos_term);

    M = A + C*sin(theta(3,2));
    N = -C*cos(theta(3,2));
    cos_term = (D1*M + H*N)/(M^2 + N^2);
    sin_term = (H - N*cos_term)/(M);
    theta(2,2) = atan2(sin_term, cos_term);

    M = A + C*sin(theta(3,3));
    N = -C*cos(theta(3,3));
    cos_term = (D2*M + H*N)/(M^2 + N^2);
    sin_term = (H - N*cos_term)/(M);
    theta(2,3) = atan2(sin_term, cos_term);

    M = A + C*sin(theta(3,4));
    N = -C*cos(theta(3,4));
    cos_term = (D2*M + H*N)/(M^2 + N^2);
    sin_term = (H - N*cos_term)/(M);
    theta(2,4) = atan2(sin_term, cos_term);


%% Joint angle 1:
% Equation:
    % y / x = tan(theta1);

% Solution
    theta(1,1) = atan2( p(2)/( lambda2 * cos( theta(2,1) ) - lambda3 * sin( theta(2,1) + theta(3,1) ) ) , p(1)/(  lambda2 * cos( theta(2,1) ) - lambda3 * sin( theta(2,1) + theta(3,1) )  ) );
    theta(1,2) = atan2( p(2)/( lambda2 * cos( theta(2,2) ) - lambda3 * sin( theta(2,2) + theta(3,2) ) ) , p(1)/(  lambda2 * cos( theta(2,2) ) - lambda3 * sin( theta(2,2) + theta(3,2) )  ) );
    theta(1,3) = atan2( p(2)/( lambda2 * cos( theta(2,3) ) - lambda3 * sin( theta(2,3) + theta(3,3) ) ) , p(1)/(  lambda2 * cos( theta(2,3) ) - lambda3 * sin( theta(2,3) + theta(3,3) )  ) );
    theta(1,4) = atan2( p(2)/( lambda2 * cos( theta(2,4) ) - lambda3 * sin( theta(2,4) + theta(3,4) ) ) , p(1)/(  lambda2 * cos( theta(2,4) ) - lambda3 * sin( theta(2,4) + theta(3,4) )  ) );
    
%% Remap theta back to phi
% phi(1) = theta(1);
% phi(2) = theta(2) - beta + pi/2;
% phi(3) = theta(3) + beta;
% phi(4) = theta(4);

phi(1,:) = theta(1,:);
phi(2,:) = theta(2,:) - beta + pi/2;
phi(3,:) = theta(3,:) + beta;
phi(4,:) = gamma;

phi = mod(phi + pi, 2*pi) - pi;

phi_optimal = phi(:,1);
if norm(phi_optimal - phi_prev) > norm(phi(:,2) - phi_prev)
    phi_optimal = phi(:,2);
end
if norm(phi_optimal - phi_prev) > norm(phi(:,3) - phi_prev)
    phi_optimal = phi(:,3);
end
if norm(phi_optimal - phi_prev) > norm(phi(:,4) - phi_prev)
    phi_optimal = phi(:,4);
end

end

== matlab function TP_CFO_Based_PP_pwm_mode/Trajectoire de référence/MATLAB Function ==
  data: pos_meas input; zone_origin input; out output; current_ input
function out = fcn(pos_meas, zone_origin, current_)

out = mod(u +1, 4);
